simulink model "SinglePhaseGridSolarPV"  (R2025b)
settings: Solver=ode23t  StartTime=0.0  StopTime=simulation.timeSim  FixedStep=0.001  MaxStep=1/(5*solarPlant.switchFrequency)  RelTol=1e-3  AbsTol=1e-3  EnableMultiTasking=on
PreLoadFcn:
  | run('SinglePhaseGridSolarPVData');
undefined symbols (not defined in the file): closedLoop, controller, grid, protection, sensor, solarPanel, solarPlant
libraries: simulink x19, fl_lib x16, nesl_utility x16, ee_lib x8, mcbeeMathTransformLib x2, simulink_extras x1, eeSinusoidalMeasurement x1, eeRmsMeasurement x1, eePwmGenerator x1
(part 2 of 2)

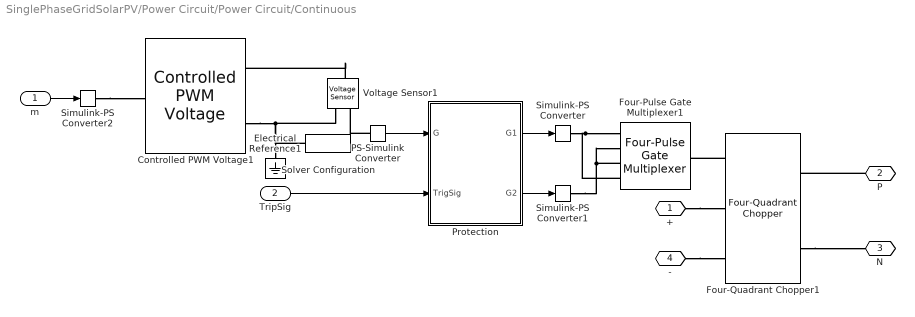
== system SinglePhaseGridSolarPV/Power Circuit/Power Circuit/Continuous ==
  m : Inport
  TripSig : Inport  Port=2
  Controlled PWM Voltage1 : ee_lib/Integrated Circuits/Controlled PWM Voltage  F=solarPlant.switchFrequency Hz  TD=0 s  pulse_width_offset=0 s  pulse_min=0 s  pwm_or_av=1  event_type=1  sample_time=1/f_pwm/100 s  Vmin=0 V  Vmax=5 V  Vm=5 V  u_min=-1  u_max=1
      settings: InternalSimscapePortConfiguration="{\"Bottom\":[],\"Left\":[{\"id\":\"u\",\"label\":\"u\",\"type\":\"input\"}],\"Right\":[{\"id\":\"p2\",\"label\":\"PWM\",\"type\":\"foundation.electrical.electrical\"},{\"id\":\"n2\",\"label\":\"REF\",\"type\":\"foundation.electrical.electrical\"}],\"Top\":[]}"
  Electrical Reference1 : fl_lib/Electrical/Electrical Elements/Electrical Reference
  Four-Pulse Gate Multiplexer1 : ee_lib/Semiconductors & Converters/Converters/Four-Pulse Gate Multiplexer  port_option=ee.enum.controlport.ps
      settings: InternalSimscapePortConfiguration="{\"Bottom\":[],\"Left\":[{\"id\":\"G1_ps\",\"label\":\"G1\",\"type\":\"input\"},{\"id\":\"G2_ps\",\"label\":\"G2\",\"type\":\"input\"},{\"id\":\"G3_ps\",\"label\":\"G3\",\"type\":\"input\"},{\"id\":\"G4_ps\",\"label\":\"G4\",\"type\":\"input\"}],\"Right\":[{\"id\":\"p\",\"label\":\"G\",\"type\":\"foundation.electrical.eight_phase\"}],\"Top\":[]}"
  Four-Quadrant Chopper1 : ee_lib/Semiconductors & Converters/Converters/Four-Quadrant Chopper  fidelity_option=ee.enum.converters.fidelity.detailed  device_type=2  showThermalPort=false  Vgt=1 V  Vgt_off=-1 V  Ih=1 A  Vf=0.8 V  Ron=0.001 Ohm  Rds=0.001 Ohm  Goff=1e-5 1/Ohm  Vth=2.5 V  K=0  Eon_scalar=22.86e-3 J  Eoff_scalar=17.14e-3 J  Eoff_natural_commutation=10e-3 J  Voff=300 V  Iout_scalar=600 A  onCurrentMeasDelay=0 s  useCurrentFromPreviousCycle=false  useVoltageFromPreviousCycle=false  diode_param=2  diode_Vf=0.8 V  diode_Ron=0.001 Ohm  diode_Goff=1e-5 1/Ohm  diode_C=50 nF  diode_iRM=-235 A  diode_iF=300 A  diode_idot=-50 A/us  diode_trr_param=1  diode_trr_factor=3  diode_trr=15 us  diode_Qrr=1500 s*uA  diode_rec_loss_model=ee.enum.diode.reverseRecoveryModel.fixed  diode_ErecVal=0 J  diode_scaleWithIandV=false  diode_ErecMat=zeros(2, 3) J  diode_TjrecVec=[298.15, 398.15] K  diode_IfrecVec=[.1, 1, 10] A  diode_IrecVal=10 A  diode_VrecVal=10 V  diode_tFilter=1 / 1000 / 100 s  thermal_network_parameterization=ee.enum.thermalNetworkTopology.external  Rth=[.08, .5] K/W  Rth_Cauer=[.08, .1, .5] K/W  Rth_Foster=[.08, .14, .22, .16] K/W  thermal_mass_parameterization=ee.enum.thermalNetwork.timeconstant  thermal_mass=[.01, .5] J/K  thermal_mass_Cauer=[.01, .1, .5] J/K  thermal_mass_Foster=[.001, .005, .05, .5] J/K  thermal_time_constant=[.001, .2] s  thermal_time_constant_Cauer=[.001, .1, .2] s  thermal_time_constant_Foster=[7e-05, .0007, .01, .08] s  thermal_mass_initial_temperatures=[25, 25] degC  thermal_mass_initial_temperatures_Cauer=[25, 25, 25] degC  junction_thermal_mass=0.01 J/K  Tvec_initial_Foster=[25, 25, 25, 25] degC  snubber_type=0  Cs=1e-7 F  Rs=0.1 Ohm
      settings: InternalSimscapePortConfiguration="{\"Bottom\":[],\"Left\":[{\"id\":\"G\",\"label\":\"G\",\"type\":\"foundation.electrical.eight_phase\"},{\"id\":\"p1\",\"label\":\"1+\",\"type\":\"foundation.electrical.electrical\"},{\"id\":\"n1\",\"label\":\"1-\",\"type\":\"foundation.electrical.electrical\"}],\"Right\":[{\"id\":\"p2\",\"label\":\"2+\",\"type\":\"foundation.electrical.electrical\"},{\"id\":\"n2\",\"label\":\"2-\",\"type\":\"foundation.electrical.electrical\"}],\"Top\":[]}"
  PS-Simulink Converter : nesl_utility/PS-Simulink Converter  PhysicalDomain=network_engine_domain  SubClassName=ps_output  LeftPortType=input  RightPortType=output  PseudoPeriodic=off  Frequencies=[]  VectorFormat=1-D array  Unit=inherit  AffineConversion=off
  Protection : Subsystem
  Simulink-PS Converter : nesl_utility/Simulink-PS Converter  PhysicalDomain=network_engine_domain  SubClassName=ps_input  LeftPortType=input  RightPortType=output  PseudoPeriodic=off  Frequencies=[]  NoiseDistribution=none  NoiseParameters=[]  Unit=1  AffineConversion=off  FilteringAndDerivatives=provide  SimscapeFilterOrder=1  InputFilterTimeConstant=0.001  UdotUserProvided=0
  Simulink-PS Converter1 : nesl_utility/Simulink-PS Converter  PhysicalDomain=network_engine_domain  SubClassName=ps_input  LeftPortType=input  RightPortType=output  PseudoPeriodic=off  Frequencies=[]  NoiseDistribution=none  NoiseParameters=[]  Unit=1  AffineConversion=off  FilteringAndDerivatives=provide  SimscapeFilterOrder=1  InputFilterTimeConstant=0.001  UdotUserProvided=0
  Simulink-PS Converter2 : nesl_utility/Simulink-PS Converter  PhysicalDomain=network_engine_domain  SubClassName=ps_input  LeftPortType=input  RightPortType=output  PseudoPeriodic=off  Frequencies=[]  NoiseDistribution=none  NoiseParameters=[]  Unit=1  AffineConversion=off  FilteringAndDerivatives=provide  SimscapeFilterOrder=1  InputFilterTimeConstant=0.001  UdotUserProvided=0
  Solver Configuration : nesl_utility/Solver Configuration  PhysicalDomain=network_engine_domain  SubClassName=solver  LeftPortType=input  RightPortType=generic  Tones=[]  Harmonics=[]  SimulateNoise=off  Profile=off  UseLocalSampling=off  EnableSwitchedLinearOptims=on  FrequencyDomain=off  UseCCode=off  RelTol=0.001  AbsTol=1e-06  MinStep=1e-09  ToWorkspace=off  RevertToSquareIcSolve=off  NumHomotopyIterations=100  PhasorMode=off  PhasorModeNumHarmonics=1  ConsistencySolver=NEWTON_FTOL  IndexReductionMethod=DerivativeReplacement  DoDC=off  ResidualTolerance=1e-09  ConsistencyTolSource=GLOBAL  ConsistencyAbsTol=0.001  ConsistencyRelTol=0.001  ConsistencyTolFactor=0.001  UseLocalSolver=off  LocalSolverChoice=NE_BACKWARD_EULER_ADVANCER  ResolveIndetEquations=on  FunctionEvalNumThread=1  LocalSolverSampleTime=0.001  DoFixedCost=off  MaxNonlinIter=3  MaxModeIter=2  ComputeImpulses=off  ImpulseIterations=2  LinearAlgebra=auto  LinearAlgebraNumThread=0  EquationFormulation=NE_TIME_EF  DelaysMemoryBudget=1024  AutomaticFiltering=on  FilteringTimeConstant=0.001  PartitionStorageMethod=AS_NEEDED  PartitionMemoryBudget=1024  PartitionMethod=ROBUST  MultibodyUseLocalSolver=off  MultibodyLocalSolverChoice=ODE1  MultibodyLocalSolverSampleTime=0.001
  Voltage Sensor1 : fl_lib/Electrical/Electrical Sensors/Voltage Sensor
  + : PMIOPort  Side=Left
  P : PMIOPort  Port=2  Side=Right
  N : PMIOPort  Port=3  Side=Right
  - : PMIOPort  Port=4  Side=Left
  wires:
  m/1 -> Simulink-PS Converter2/1
  PS-Simulink Converter/1 -> Protection/1(G)
  Protection/1(G1) -> Simulink-PS Converter/1
  Protection/2(G2) -> Simulink-PS Converter1/1
  TripSig/1 -> Protection/2(TrigSig)
  connections:
  Voltage Sensor1/LConn1 -- Controlled PWM Voltage1/RConn1
  Controlled PWM Voltage1/RConn2 -- Solver Configuration/RConn1 -- Electrical Reference1/LConn1 -- Voltage Sensor1/RConn2
  Simulink-PS Converter2/RConn1 -- Controlled PWM Voltage1/LConn1
  PS-Simulink Converter/LConn1 -- Voltage Sensor1/RConn1
  P/RConn1 -- Four-Quadrant Chopper1/RConn1
  Four-Pulse Gate Multiplexer1/LConn4 -- Four-Pulse Gate Multiplexer1/LConn1 -- Simulink-PS Converter/RConn1
  Four-Quadrant Chopper1/RConn2 -- N/RConn1
  Four-Pulse Gate Multiplexer1/LConn3 -- Four-Pulse Gate Multiplexer1/LConn2 -- Simulink-PS Converter1/RConn1
  +/RConn1 -- Four-Quadrant Chopper1/LConn2
  -/RConn1 -- Four-Quadrant Chopper1/LConn3
  Four-Quadrant Chopper1/LConn1 -- Four-Pulse Gate Multiplexer1/RConn1

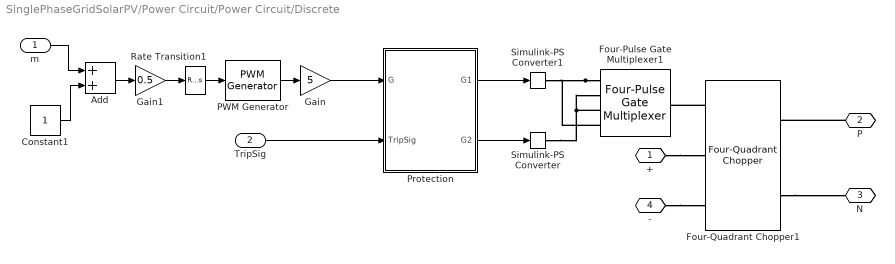
== system SinglePhaseGridSolarPV/Power Circuit/Power Circuit/Discrete ==
  m : Inport
  TripSig : Inport  Port=2
  Add : Sum
  Constant1 : Constant
  Four-Pulse Gate Multiplexer1 : ee_lib/Semiconductors & Converters/Converters/Four-Pulse Gate Multiplexer  port_option=ee.enum.controlport.ps
      settings: InternalSimscapePortConfiguration="{\"Bottom\":[],\"Left\":[{\"id\":\"G1_ps\",\"label\":\"G1\",\"type\":\"input\"},{\"id\":\"G2_ps\",\"label\":\"G2\",\"type\":\"input\"},{\"id\":\"G3_ps\",\"label\":\"G3\",\"type\":\"input\"},{\"id\":\"G4_ps\",\"label\":\"G4\",\"type\":\"input\"}],\"Right\":[{\"id\":\"p\",\"label\":\"G\",\"type\":\"foundation.electrical.eight_phase\"}],\"Top\":[]}"
  Four-Quadrant Chopper1 : ee_lib/Semiconductors & Converters/Converters/Four-Quadrant Chopper  fidelity_option=ee.enum.converters.fidelity.detailed  device_type=2  showThermalPort=false  Vgt=1 V  Vgt_off=-1 V  Ih=1 A  Vf=0.8 V  Ron=0.001 Ohm  Rds=0.001 Ohm  Goff=1e-5 1/Ohm  Vth=2.5 V  K=0  Eon_scalar=22.86e-3 J  Eoff_scalar=17.14e-3 J  Eoff_natural_commutation=10e-3 J  Voff=300 V  Iout_scalar=600 A  onCurrentMeasDelay=0 s  useCurrentFromPreviousCycle=false  useVoltageFromPreviousCycle=false  diode_param=2  diode_Vf=0.8 V  diode_Ron=0.001 Ohm  diode_Goff=1e-5 1/Ohm  diode_C=50 nF  diode_iRM=-235 A  diode_iF=300 A  diode_idot=-50 A/us  diode_trr_param=1  diode_trr_factor=3  diode_trr=15 us  diode_Qrr=1500 s*uA  diode_rec_loss_model=ee.enum.diode.reverseRecoveryModel.fixed  diode_ErecVal=0 J  diode_scaleWithIandV=false  diode_ErecMat=zeros(2, 3) J  diode_TjrecVec=[298.15, 398.15] K  diode_IfrecVec=[.1, 1, 10] A  diode_IrecVal=10 A  diode_VrecVal=10 V  diode_tFilter=1 / 1000 / 100 s  thermal_network_parameterization=ee.enum.thermalNetworkTopology.external  Rth=[.08, .5] K/W  Rth_Cauer=[.08, .1, .5] K/W  Rth_Foster=[.08, .14, .22, .16] K/W  thermal_mass_parameterization=ee.enum.thermalNetwork.timeconstant  thermal_mass=[.01, .5] J/K  thermal_mass_Cauer=[.01, .1, .5] J/K  thermal_mass_Foster=[.001, .005, .05, .5] J/K  thermal_time_constant=[.001, .2] s  thermal_time_constant_Cauer=[.001, .1, .2] s  thermal_time_constant_Foster=[7e-05, .0007, .01, .08] s  thermal_mass_initial_temperatures=[25, 25] degC  thermal_mass_initial_temperatures_Cauer=[25, 25, 25] degC  junction_thermal_mass=0.01 J/K  Tvec_initial_Foster=[25, 25, 25, 25] degC  snubber_type=0  Cs=1e-7 F  Rs=0.1 Ohm
      settings: InternalSimscapePortConfiguration="{\"Bottom\":[],\"Left\":[{\"id\":\"G\",\"label\":\"G\",\"type\":\"foundation.electrical.eight_phase\"},{\"id\":\"p1\",\"label\":\"1+\",\"type\":\"foundation.electrical.electrical\"},{\"id\":\"n1\",\"label\":\"1-\",\"type\":\"foundation.electrical.electrical\"}],\"Right\":[{\"id\":\"p2\",\"label\":\"2+\",\"type\":\"foundation.electrical.electrical\"},{\"id\":\"n2\",\"label\":\"2-\",\"type\":\"foundation.electrical.electrical\"}],\"Top\":[]}"
  Gain : Gain  Gain=5
  Gain1 : Gain  Gain=0.5
  PWM Generator : eePwmGenerator/PWM Generator  CarrCount=Up  Tper=1/solarPlant.switchFrequency  Tdelay=0  Ts=1/(10*solarPlant.switchFrequency)
  Protection : Subsystem
  Rate Transition1 : RateTransition  OutPortSampleTime=1/(10*solarPlant.switchFrequency)
  Simulink-PS Converter : nesl_utility/Simulink-PS Converter  PhysicalDomain=network_engine_domain  SubClassName=ps_input  LeftPortType=input  RightPortType=output  PseudoPeriodic=off  Frequencies=[]  NoiseDistribution=none  NoiseParameters=[]  Unit=1  AffineConversion=off  FilteringAndDerivatives=provide  SimscapeFilterOrder=1  InputFilterTimeConstant=0.001  UdotUserProvided=0
  Simulink-PS Converter1 : nesl_utility/Simulink-PS Converter  PhysicalDomain=network_engine_domain  SubClassName=ps_input  LeftPortType=input  RightPortType=output  PseudoPeriodic=off  Frequencies=[]  NoiseDistribution=none  NoiseParameters=[]  Unit=1  AffineConversion=off  FilteringAndDerivatives=provide  SimscapeFilterOrder=1  InputFilterTimeConstant=0.001  UdotUserProvided=0
  + : PMIOPort  Side=Left
  P : PMIOPort  Port=2  Side=Right
  N : PMIOPort  Port=3  Side=Right
  - : PMIOPort  Port=4  Side=Left
  wires:
  Constant1/1 -> Add/2
  Rate Transition1/1 -> PWM Generator/1
  m/1 -> Add/1
  Gain1/1 -> Rate Transition1/1
  PWM Generator/1 -> Gain/1
  Add/1 -> Gain1/1
  Protection/1(G1) -> Simulink-PS Converter1/1
  Protection/2(G2) -> Simulink-PS Converter/1
  Gain/1 -> Protection/1(G)
  TripSig/1 -> Protection/2(TripSig)
  connections:
  Four-Pulse Gate Multiplexer1/LConn3 -- Four-Pulse Gate Multiplexer1/LConn2 -- Simulink-PS Converter/RConn1
  P/RConn1 -- Four-Quadrant Chopper1/RConn1
  Four-Pulse Gate Multiplexer1/LConn1 -- Four-Pulse Gate Multiplexer1/LConn4 -- Simulink-PS Converter1/RConn1
  Four-Quadrant Chopper1/RConn2 -- N/RConn1
  -/RConn1 -- Four-Quadrant Chopper1/LConn3
  Four-Quadrant Chopper1/LConn1 -- Four-Pulse Gate Multiplexer1/RConn1
  +/RConn1 -- Four-Quadrant Chopper1/LConn2

== system SinglePhaseGridSolarPV/MPPT/MPPT Algorithm/IncrementalConductance/If Action Subsystem ==
  In1 : Inport
  Action Port : ActionPort  ActionPortLabel=if(u1 == 0)
  Compare To Constant : simulink/Logic and Bit Operations/Compare To Constant  relop===  const=0  OutDataTypeStr=boolean
  Compare To Zero2 : simulink/Logic and Bit Operations/Compare To Zero  relop=>  OutDataTypeStr=boolean
  Set : Outport  VectorParamsAs1DForOutWhenUnconnected=off
  Inc : Outport  Port=2  VectorParamsAs1DForOutWhenUnconnected=off
  wires:
  Compare To Constant/1 -> Set/1  "Yes"
  Compare To Zero2/1 -> Inc/1  "Yes"
  In1/1 -> Compare To Zero2/1, Compare To Constant/1  "delI"

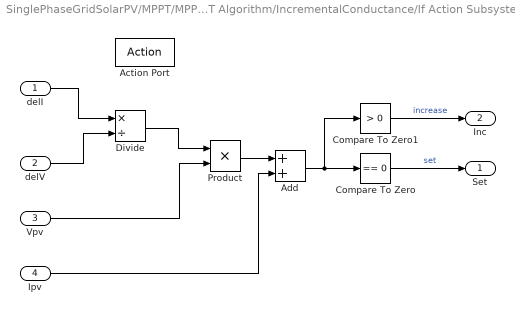
== system SinglePhaseGridSolarPV/MPPT/MPPT Algorithm/IncrementalConductance/If Action Subsystem1 ==
  delI : Inport
  delV : Inport  Port=2
  Vpv : Inport  Port=3
  Ipv : Inport  Port=4
  Action Port : ActionPort  ActionPortLabel=else
  Add : Sum
  Compare To Zero : simulink/Logic and Bit Operations/Compare To Zero  relop===  OutDataTypeStr=boolean
  Compare To Zero1 : simulink/Logic and Bit Operations/Compare To Zero  relop=>  OutDataTypeStr=boolean
  Divide : Product  Inputs=*/
  Product : Product
  Set : Outport  VectorParamsAs1DForOutWhenUnconnected=off
  Inc : Outport  Port=2  VectorParamsAs1DForOutWhenUnconnected=off
  wires:
  delI/1 -> Divide/1
  delV/1 -> Divide/2
  Divide/1 -> Product/1
  Add/1 -> Compare To Zero1/1, Compare To Zero/1
  Compare To Zero1/1 -> Inc/1  "increase"
  Compare To Zero/1 -> Set/1  "set"
  Vpv/1 -> Product/2
  Product/1 -> Add/1
  Ipv/1 -> Add/2

== system SinglePhaseGridSolarPV/Power Circuit/Power Circuit/Average/Map [-1,1] to [0,1] ==
  PS Add : fl_lib/Physical Signals/Functions/PS Add
  PS Constant : fl_lib/Physical Signals/Sources/PS Constant  constant=1
  PS Gain : fl_lib/Physical Signals/Functions/PS Gain  gain=0.5
  u : PMIOPort  Side=Left
  y : PMIOPort  Port=2  Side=Right
  connections:
  PS Constant/RConn1 -- PS Add/LConn1
  PS Gain/RConn1 -- y/RConn1
  PS Add/RConn1 -- PS Gain/LConn1
  u/RConn1 -- PS Add/LConn2

== system SinglePhaseGridSolarPV/Power Circuit/Power Circuit/Continuous/Protection ==
  G : Inport
  TrigSig : Inport  Port=2
  Constant : Constant  Value=5
  Constant2 : Constant  Value=0
  NOT : Logic  Operator=NOT  IconShape=distinctive  AllPortsSameDT=off  OutDataTypeStr=boolean
  Subtract : Sum  Inputs=-+
  Switch : Switch  Criteria=u2 > Threshold  SaturateOnIntegerOverflow=off  InputSameDT=off
  Switch1 : Switch  Criteria=u2 > Threshold  SaturateOnIntegerOverflow=off  InputSameDT=off
  G1 : Outport  VectorParamsAs1DForOutWhenUnconnected=off
  G2 : Outport  Port=2  VectorParamsAs1DForOutWhenUnconnected=off
  wires:
  Switch1/1 -> G2/1
  NOT/1 -> Switch/2
  Constant2/1 -> Switch/3, Switch1/1
  Constant/1 -> Subtract/2
  Switch/1 -> G1/1
  Subtract/1 -> Switch1/3
  G/1 -> Switch/1, Subtract/1
  TrigSig/1 -> Switch1/2, NOT/1

== system SinglePhaseGridSolarPV/Power Circuit/Power Circuit/Discrete/Protection ==
  G : Inport
  TripSig : Inport  Port=2
  Constant : Constant  Value=5
  Constant2 : Constant  Value=0
  NOT : Logic  Operator=NOT  IconShape=distinctive  AllPortsSameDT=off  OutDataTypeStr=boolean
  Subtract : Sum  Inputs=-+
  Switch : Switch  Criteria=u2 > Threshold  SaturateOnIntegerOverflow=off  InputSameDT=off
  Switch1 : Switch  Criteria=u2 > Threshold  SaturateOnIntegerOverflow=off  InputSameDT=off
  G1 : Outport  VectorParamsAs1DForOutWhenUnconnected=off
  G2 : Outport  Port=2  VectorParamsAs1DForOutWhenUnconnected=off
  wires:
  Switch1/1 -> G2/1
  NOT/1 -> Switch/2
  Constant2/1 -> Switch/3, Switch1/1
  Constant/1 -> Subtract/2
  Switch/1 -> G1/1
  Subtract/1 -> Switch1/3
  G/1 -> Switch/1, Subtract/1
  TripSig/1 -> Switch1/2, NOT/1
